simulink library "casper_library_communications"  (R2021a)
settings: Solver=ode45  StartTime=0.0  StopTime=10.0  RelTol=1e-3
undefined symbols (not defined in the file or in its folder): Down, Up
libraries: xbsIndex_r4 x292, casper_library_misc x6, xbsReplacements_r4 x6, xps_library x2
(part 1 of 2)
settings Model: Creator=mdexter  LastModifiedBy=jkocz
settings SolverCC: AlgebraicLoopSolver=TrustRegion
settings DataIOCC: LimitDataPoints=on  SaveFormat=Array  SignalLoggingSaveFormat=ModelDataLogs  ReturnWorkspaceOutputs=off
settings OptimizationCC: BlockReduction=off  BooleanDataType=off  ExpressionDepthLimit=2147483647  LifeSpan=inf
settings DebuggingCC: SaveWithParameterizedLinksMsg=none  UnderspecifiedInitializationDetection=Classic  MergeDetectMultiDrivingBlocksExec=none  SignalResolutionControl=TryResolveAllWithWarning  FcnCallInpInsideContextMsg=warning  StateNameClashWarn=warning  SFUnexpectedBacktrackingDiag=warning  SFNoUnconditionalDefaultTransitionDiag=warning  SFExecutionAtInitializationDiag=none  SFMachineParentedDataDiag=warning  ArithmeticOperatorsInVariantConditions=warning
settings HardwareCC: ProdBitPerPointer=32  ProdBitPerSizeT=32  ProdBitPerPtrDiffT=32  ProdLargestAtomicFloat=None  ProdIntDivRoundTo=Undefined  ProdEndianess=Unspecified  ProdWordSize=32  ProdHWDeviceType=32-bit Generic  TargetUnknown=on
settings ModelReferenceCC: PropagateSignalLabelsOutOfModel=off
settings SFSimCC: SimUseLocalCustomCode=off  CustomCodeUndefinedFunction=UseInterfaceOnly
settings RTWCC: RTWUseLocalCustomCode=off
settings CodeAppCC: StateflowObjectComments=on
settings GRTTargetCC: TargetLangStandard=C89/C90 (ANSI)  CombineOutputUpdateFcns=off  GRTInterface=on
settings ConfigComp: CovMetricSettings=dw  CovSaveCumulativeToWorkspaceVar=on  CovSaveSingleToWorkspaceVar=on  CovExternalEMLEnable=off

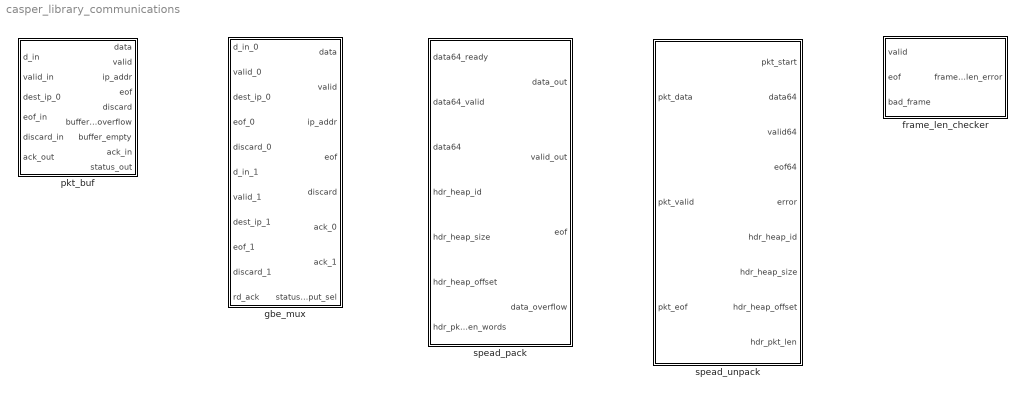
== system casper_library_communications ==
  frame_len_checker : Subsystem  Tag=casper:frame_len_checker  mask{frame_len=640 + 3 + 1}
      mask prompts: frame_len "Frame length (64-bit words):"
      mask help: Monitors valid, EOF and bad_frame signals in/from a 10Gbe core and outputs an error signal. Can be used to drive an error counter or latched as a flag.
  gbe_mux : Subsystem  mask(pkt_mux){}
      mask help: Merges two packet streams into one. Does round-robin arbitration.
  pkt_buf : Subsystem  mask(mux_packets){depth_data_bits=10, depth_hdr_bits=5}
      mask prompts: depth_data_bits "Depth contents (2^?)"; depth_hdr_bits "Maximum number of packets to buffer? (2^?)"
      mask help: This block allows you to buffer a 10GbE datastream.
      mask init:
      | fmtstr = sprintf('Max %d data words.\nMax %d pkts.', 2^depth_data_bits,2^depth_hdr_bits);
      | set_param(gcb, 'AttributesFormatString', fmtstr);
      settings: AttributesFormatString=|
      | Max 1024 data words.
      | Max 32 pkts.
  spead_pack : Subsystem  Tag=casper:spead_pack  mask(pkt_pack_mask){max_pkt_len_bits=10, header_ids=0x1600, 0x1234, header_ind_ids=0x1800, spead_msw=64, spead_lsw=40, spead_version=4, bytes_per_word=8}
      mask prompts: max_pkt_len_bits "Max pkt length, 2^? 64-bit words"; header_ids "SPEAD direct address IDs (decimal)"; header_ind_ids "SPEAD indirect address IDs (decimal)"; spead_msw "SPEAD Flavour (MSw)"; spead_lsw "SPEAD Flavour (LSw)"; spead_version "SPEAD version"; bytes_per_word "Word size, in bytes"
      mask help:
      | This block generates SPEAD-compliant packets from a datastream.
      |
      | Packets are created with a fixed header followed by a number of 64-bit items.
      |
      | Requires a 64-bit data stream.
      |
      | The data_ready signal is one cycle BEFORE valid data! Does not have to be with a valid signal either.
      mask init:
      | if floor(log2(bytes_per_word)) ~= log2(bytes_per_word)
      |     error('Bytes per word should be a power of two.');
      | end
      | 
      | spead_pack_init(gcb)
  spead_unpack : Subsystem  Tag=casper:spead_unpack  mask(spead_unpack_mask){max_pkt_len_bits=10, header_ids=0x1600, 0x1234, header_ind_ids=0x1800, spead_msw=64, spead_lsw=40, spead_version=4, combine_errors=on}
      mask prompts: max_pkt_len_bits "Max pkt length, 2^? 64-bit words"; header_ids "SPEAD direct header IDs (decimal)"; header_ind_ids "SPEAD indirect address IDs (decimal)"; spead_msw "SPEAD Flavour (MSw)"; spead_lsw "SPEAD Flavour (LSw)"; spead_version "SPEAD version"; combine_errors "Combine error flags"
      mask help: This block receives a 64-bit-word stream that contains a SPEAD stream. It checks the SPEAD headers are being correctly received. It presents the user with all headers on the first valid cycle of data along with a flag to indicate a header or packet-length error.
      mask init:
      | spead_unpack_init(gcb)

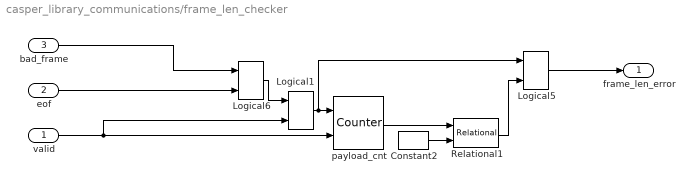
== system casper_library_communications/frame_len_checker ==
  valid : Inport
  eof : Inport  Port=2
  bad_frame : Inport  Port=3
  Constant2 : xbsIndex_r4/Constant  const=frame_len - 1  gui_display_data_type=Fixed-point  arith_type=Unsigned  n_bits=(ceil(log2(frame_len)))+1  bin_pt=0  preci_type=Single  exp_width=8  frac_width=24  explicit_period=on  period=1  equ=P=C  opselect=C  inp2=PCIN>>17  opr=+  inp1=P  carry=CIN  dbl_ovrd=off  block_type=constant
  Logical1 : xbsIndex_r4/Logical  logical_function=AND  inputs=2  en=off  latency=0  precision=Full  arith_type=Unsigned  n_bits=8  bin_pt=2  align_bp=on  dbl_ovrd=off  block_type=logical
      settings: xl_area=[0, 0, 0, 0, 0, 0, 0]
  Logical5 : xbsIndex_r4/Logical  logical_function=AND  inputs=2  en=off  latency=0  precision=Full  arith_type=Unsigned  n_bits=8  bin_pt=2  align_bp=on  dbl_ovrd=off  block_type=logical
      settings: xl_area=[0, 0, 0, 0, 0, 0, 0]
  Logical6 : xbsIndex_r4/Logical  logical_function=OR  inputs=2  en=off  latency=0  precision=Full  arith_type=Unsigned  n_bits=8  bin_pt=2  align_bp=on  dbl_ovrd=off  block_type=logical
      settings: xl_area=[0, 0, 0, 0, 0, 0, 0]
  Relational1 : xbsIndex_r4/Relational  mode=a!=b  op_type=Bool  en=off  latency=0  dbl_ovrd=off  block_type=relational
      settings: xl_area=[0, 0, 0, 0, 0, 0, 0]  block_version=10.1.3
  payload_cnt : xbsIndex_r4/Counter  cnt_type=Free Running  cnt_to=frame_len - 1  operation=Up  start_count=0  cnt_by_val=1  arith_type=Unsigned  n_bits=(ceil(log2(frame_len)))+1  bin_pt=0  load_pin=off  rst=on  en=on  explicit_period=off  period=1  use_behavioral_HDL=off  implementation=Fabric  use_rpm=on  dbl_ovrd=off  block_type=counter
      settings: xl_area=[0, 0, 0, 0, 0, 0, 0]
  frame_len_error : Outport  VectorParamsAs1DForOutWhenUnconnected=off
  wires:
  Logical1/1 -> Logical5/1, payload_cnt/1
  eof/1 -> Logical6/2
  Relational1/1 -> Logical5/2
  payload_cnt/1 -> Relational1/1
  Constant2/1 -> Relational1/2
  bad_frame/1 -> Logical6/1
  valid/1 -> Logical1/2, payload_cnt/2
  Logical6/1 -> Logical1/1
  Logical5/1 -> frame_len_error/1

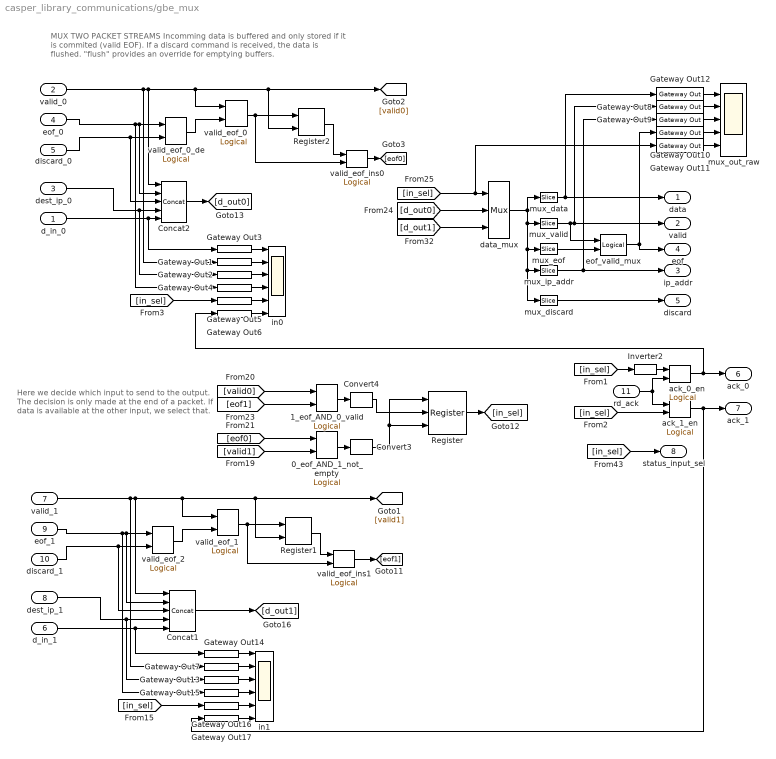
== system casper_library_communications/gbe_mux ==
  note: MUX TWO PACKET STREAMS
      | Incomming data is buffered and only stored if it is commited (valid EOF).
      | If a discard command is received, the data is flushed.
      | "flush" provides an override for emptying buffers.
  note: Here we decide which input
      | to send to the output.
      | The decision is only made at the end of a packet.
      | If data is available at the other input,
      | we select that.
  d_in_0 : Inport
  valid_0 : Inport  Port=2
  dest_ip_0 : Inport  Port=3
  eof_0 : Inport  Port=4
  discard_0 : Inport  Port=5
  d_in_1 : Inport  Port=6
  valid_1 : Inport  Port=7
  dest_ip_1 : Inport  Port=8
  eof_1 : Inport  Port=9
  discard_1 : Inport  Port=10
  rd_ack : Inport  Port=11
  0_eof_AND_1_not_empty : xbsIndex_r4/Logical  logical_function=AND  inputs=2  en=off  latency=0  precision=Full  arith_type=Unsigned  n_bits=8  bin_pt=2  align_bp=on  dbl_ovrd=off  block_type=logical
      settings: xl_area=[0, 0, 0, 0, 0, 0, 0]
  1_eof_AND_0_valid : xbsIndex_r4/Logical  logical_function=AND  inputs=2  en=off  latency=0  precision=Full  arith_type=Unsigned  n_bits=8  bin_pt=2  align_bp=on  dbl_ovrd=off  block_type=logical
      settings: xl_area=[0, 0, 0, 0, 0, 0, 0]
  Concat1 : xbsIndex_r4/Concat  num_inputs=5  dbl_ovrd=off  block_type=concat
      settings: block_version=10.1.3
  Concat2 : xbsIndex_r4/Concat  num_inputs=5  dbl_ovrd=off  block_type=concat
      settings: block_version=10.1.3
  Convert3 : xbsIndex_r4/Convert  gui_display_data_type=Fixed-point  arith_type=Boolean  n_bits=8  bin_pt=6  float_type=Single  exp_bits=8  fraction_bits=24  quantization=Truncate  overflow=Wrap  en=off  latency=0  pipeline=off  dbl_ovrd=off  block_type=convert
      settings: xl_area=[0, 0, 0, 0, 0, 0, 0]  block_version=10.1.3
  Convert4 : xbsIndex_r4/Convert  gui_display_data_type=Fixed-point  arith_type=Boolean  n_bits=8  bin_pt=6  float_type=Single  exp_bits=8  fraction_bits=24  quantization=Truncate  overflow=Wrap  en=off  latency=0  pipeline=off  dbl_ovrd=off  block_type=convert
      settings: xl_area=[0, 0, 0, 0, 0, 0, 0]  block_version=10.1.3
  Gateway Out{1..17} (17 alike) : xbsIndex_r4/Gateway Out  inherit_from_input=off  hdl_port=off  rows=1  columns=1  UseAsDAC=off  DACChannel='1'  interface=None  automatic_assignment=on  address_offset=hex2dec('00')  intf_name=''  intf_description=''  timing_constraint=None  locs_specified=off  LOCs={}  io_standard={}  block_type=gatewayout
      settings: infoedit="Gateway out block.  Converts Xilinx fixed point inputs into ouputs of type Simulink integer, double, or fixed point.<P><P>Hardware notes:  In hardware these blocks become top level output ports or are discarded, depending on how they are configured."  xl_area=[0, 0, 0, 0, 0, 0, 0]  block_version=10.1.3
  Inverter2 : xbsIndex_r4/Inverter  en=off  latency=0  dbl_ovrd=off  block_type=inv
      settings: xl_area=[0, 0, 0, 0, 0, 0, 0]
  Register : xbsIndex_r4/Register  init=0  rst=on  en=on  dbl_ovrd=off  block_type=register
      settings: xl_area=[0, 0, 0, 0, 0, 0, 0]
  Register1 : xbsIndex_r4/Register  init=1  rst=off  en=on  dbl_ovrd=off  block_type=register
      settings: xl_area=[0, 0, 0, 0, 0, 0, 0]
  Register2 : xbsIndex_r4/Register  init=0  rst=off  en=on  dbl_ovrd=off  block_type=register
      settings: xl_area=[0, 0, 0, 0, 0, 0, 0]
  ack_0_en : xbsIndex_r4/Logical  logical_function=AND  inputs=2  en=off  latency=0  precision=Full  arith_type=Unsigned  n_bits=8  bin_pt=2  align_bp=on  dbl_ovrd=off  block_type=logical
      settings: xl_area=[0, 0, 0, 0, 0, 0, 0]
  ack_1_en : xbsIndex_r4/Logical  logical_function=AND  inputs=2  en=off  latency=0  precision=Full  arith_type=Unsigned  n_bits=8  bin_pt=2  align_bp=on  dbl_ovrd=off  block_type=logical
      settings: xl_area=[0, 0, 0, 0, 0, 0, 0]
  data_mux : xbsIndex_r4/Mux  inputs=2  en=off  latency=0  precision=Full  arith_type="Signed  (2's comp)"  n_bits=8  bin_pt=2  quantization=Truncate  overflow=Wrap  dbl_ovrd=off  block_type=mux
      settings: xl_area=[0, 0, 0, 0, 0, 0, 0]
  eof_valid_mux : xbsIndex_r4/Logical  logical_function=AND  inputs=2  en=off  latency=0  precision=Full  arith_type=Unsigned  n_bits=8  bin_pt=2  align_bp=on  dbl_ovrd=off  block_type=logical
      settings: xl_area=[0, 0, 0, 0, 0, 0, 0]
  in0 : Scope  NumInputPorts=6
  in1 : Scope  NumInputPorts=6
  mux_data : xbsIndex_r4/Slice  nbits=64  boolean_output=off  mode=Lower Bit Location + Width  bit1=33  base1=LSB of Input  bit0=0  base0=LSB of Input  dbl_ovrd=off  block_type=slice
      settings: infoedit="Extracts a given range of bits from each input sample and presents it at the output.  The output type is ordinarily unsigned with binary point at zero, but can be Boolean when the slice is one bit wide.<P><P>Hardware notes: In hardware this block costs nothing."  block_version=10.1.3
  mux_discard : xbsIndex_r4/Slice  nbits=1  boolean_output=on  mode=Lower Bit Location + Width  bit1=0  base1=MSB of Input  bit0=96  base0=LSB of Input  dbl_ovrd=off  block_type=slice
      settings: infoedit="Extracts a given range of bits from each input sample and presents it at the output.  The output type is ordinarily unsigned with binary point at zero, but can be Boolean when the slice is one bit wide.<P><P>Hardware notes: In hardware this block costs nothing."  block_version=10.1.3
  mux_eof : xbsIndex_r4/Slice  nbits=1  boolean_output=on  mode=Upper Bit Location + Width  bit1=97  base1=LSB of Input  bit0=0  base0=LSB of Input  dbl_ovrd=off  block_type=slice
      settings: infoedit="Extracts a given range of bits from each input sample and presents it at the output.  The output type is ordinarily unsigned with binary point at zero, but can be Boolean when the slice is one bit wide.<P><P>Hardware notes: In hardware this block costs nothing."  block_version=10.1.3
  mux_ip_addr : xbsIndex_r4/Slice  nbits=32  boolean_output=off  mode=Lower Bit Location + Width  bit1=0  base1=MSB of Input  bit0=64  base0=LSB of Input  dbl_ovrd=off  block_type=slice
      settings: infoedit="Extracts a given range of bits from each input sample and presents it at the output.  The output type is ordinarily unsigned with binary point at zero, but can be Boolean when the slice is one bit wide.<P><P>Hardware notes: In hardware this block costs nothing."  block_version=10.1.3
  mux_out_raw : Scope  NumInputPorts=5
  mux_valid : xbsIndex_r4/Slice  nbits=1  boolean_output=on  mode=Lower Bit Location + Width  bit1=0  base1=MSB of Input  bit0=98  base0=LSB of Input  dbl_ovrd=off  block_type=slice
      settings: infoedit="Extracts a given range of bits from each input sample and presents it at the output.  The output type is ordinarily unsigned with binary point at zero, but can be Boolean when the slice is one bit wide.<P><P>Hardware notes: In hardware this block costs nothing."  block_version=10.1.3
  valid_eof_0 : xbsIndex_r4/Logical  logical_function=AND  inputs=2  en=off  latency=0  precision=Full  arith_type=Unsigned  n_bits=8  bin_pt=2  align_bp=on  dbl_ovrd=off  block_type=logical
      settings: xl_area=[0, 0, 0, 0, 0, 0, 0]
  valid_eof_0_de : xbsIndex_r4/Logical  logical_function=OR  inputs=2  en=off  latency=0  precision=Full  arith_type=Unsigned  n_bits=8  bin_pt=2  align_bp=on  dbl_ovrd=off  block_type=logical
      settings: xl_area=[0, 0, 0, 0, 0, 0, 0]
  valid_eof_1 : xbsIndex_r4/Logical  logical_function=AND  inputs=2  en=off  latency=0  precision=Full  arith_type=Unsigned  n_bits=8  bin_pt=2  align_bp=on  dbl_ovrd=off  block_type=logical
      settings: xl_area=[0, 0, 0, 0, 0, 0, 0]
  valid_eof_2 : xbsIndex_r4/Logical  logical_function=OR  inputs=2  en=off  latency=0  precision=Full  arith_type=Unsigned  n_bits=8  bin_pt=2  align_bp=on  dbl_ovrd=off  block_type=logical
      settings: xl_area=[0, 0, 0, 0, 0, 0, 0]
  valid_eof_ins0 : xbsIndex_r4/Logical  logical_function=OR  inputs=2  en=off  latency=0  precision=Full  arith_type=Unsigned  n_bits=8  bin_pt=2  align_bp=on  dbl_ovrd=off  block_type=logical
      settings: xl_area=[0, 0, 0, 0, 0, 0, 0]
  valid_eof_ins1 : xbsIndex_r4/Logical  logical_function=OR  inputs=2  en=off  latency=0  precision=Full  arith_type=Unsigned  n_bits=8  bin_pt=2  align_bp=on  dbl_ovrd=off  block_type=logical
      settings: xl_area=[0, 0, 0, 0, 0, 0, 0]
  data : Outport  VectorParamsAs1DForOutWhenUnconnected=off
  valid : Outport  Port=2  VectorParamsAs1DForOutWhenUnconnected=off
  ip_addr : Outport  Port=3  VectorParamsAs1DForOutWhenUnconnected=off
  eof : Outport  Port=4  VectorParamsAs1DForOutWhenUnconnected=off
  discard : Outport  Port=5  VectorParamsAs1DForOutWhenUnconnected=off
  ack_0 : Outport  Port=6  VectorParamsAs1DForOutWhenUnconnected=off
  ack_1 : Outport  Port=7  VectorParamsAs1DForOutWhenUnconnected=off
  status_input_sel : Outport  Port=8  VectorParamsAs1DForOutWhenUnconnected=off
  wires:
  valid_eof_ins0/1 -> [eof0]
  Register2/1 -> valid_eof_ins0/1
  Register1/1 -> valid_eof_ins1/1
  valid_eof_ins1/1 -> [eof1]
  Gateway Out17/1 -> in1/6
  Gateway Out6/1 -> in0/6
  mux_discard/1 -> discard/1
  d_in_0/1 -> Concat2/5, Gateway Out3/1
  dest_ip_0/1 -> Gateway Out2/1, Concat2/4
  valid_eof_0_de/1 -> valid_eof_0/2
  discard_0/1 -> Concat2/3, valid_eof_0_de/2
  eof_0/1 -> Gateway Out4/1, Concat2/2, valid_eof_0_de/1
  Gateway Out5/1 -> in0/5
  [in_sel] -> Gateway Out5/1
  Gateway Out4/1 -> in0/4
  Gateway Out2/1 -> in0/3
  Gateway Out1/1 -> in0/2
  Gateway Out3/1 -> in0/1
  Concat2/1 -> [d_out0]
  valid_eof_0/1 -> valid_eof_ins0/2, Register2/1
  valid_0/1 -> Gateway Out1/1, Concat2/1, [valid0], Register2/2, valid_eof_0/1
  d_in_1/1 -> Gateway Out14/1, Concat1/5
  dest_ip_1/1 -> Gateway Out13/1, Concat1/4
  [in_sel] -> Inverter2/1
  Inverter2/1 -> ack_0_en/1
  [in_sel] -> ack_1_en/2
  rd_ack/1 -> ack_1_en/1, ack_0_en/2
  ack_1_en/1 -> Gateway Out17/1, ack_1/1
  ack_0_en/1 -> Gateway Out6/1, ack_0/1
  valid_eof_2/1 -> valid_eof_1/2
  discard_1/1 -> Concat1/3, valid_eof_2/2
  eof_1/1 -> Gateway Out15/1, Concat1/2, valid_eof_2/1
  Gateway Out16/1 -> in1/5
  [in_sel] -> Gateway Out16/1
  Register/1 -> [in_sel]
  Gateway Out11/1 -> mux_out_raw/5
  Gateway Out15/1 -> in1/4
  Gateway Out13/1 -> in1/3
  Gateway Out7/1 -> in1/2
  Gateway Out14/1 -> in1/1
  mux_eof/1 -> eof_valid_mux/2
  eof_valid_mux/1 -> Gateway Out10/1, eof/1
  mux_ip_addr/1 -> Gateway Out9/1, ip_addr/1
  mux_valid/1 -> Gateway Out8/1, valid/1, eof_valid_mux/1
  mux_data/1 -> data/1, Gateway Out12/1
  data_mux/1 -> mux_data/1, mux_valid/1, mux_eof/1, mux_discard/1, mux_ip_addr/1
  Concat1/1 -> [d_out1]
  valid_eof_1/1 -> valid_eof_ins1/2, Register1/1
  [in_sel] -> status_input_sel/1
  [d_out1] -> data_mux/3
  [d_out0] -> data_mux/2
  [in_sel] -> Gateway Out11/1, data_mux/1
  [eof1] -> 1_eof_AND_0_valid/2
  [eof0] -> 0_eof_AND_1_not_empty/1
  [valid0] -> 1_eof_AND_0_valid/1
  [valid1] -> 0_eof_AND_1_not_empty/2
  Gateway Out10/1 -> mux_out_raw/4
  Gateway Out9/1 -> mux_out_raw/3
  Gateway Out8/1 -> mux_out_raw/2
  Gateway Out12/1 -> mux_out_raw/1
  Convert4/1 -> Register/2
  Convert3/1 -> Register/1, Register/3
  1_eof_AND_0_valid/1 -> Convert4/1
  0_eof_AND_1_not_empty/1 -> Convert3/1
  valid_1/1 -> Gateway Out7/1, Concat1/1, [valid1], Register1/2, valid_eof_1/1

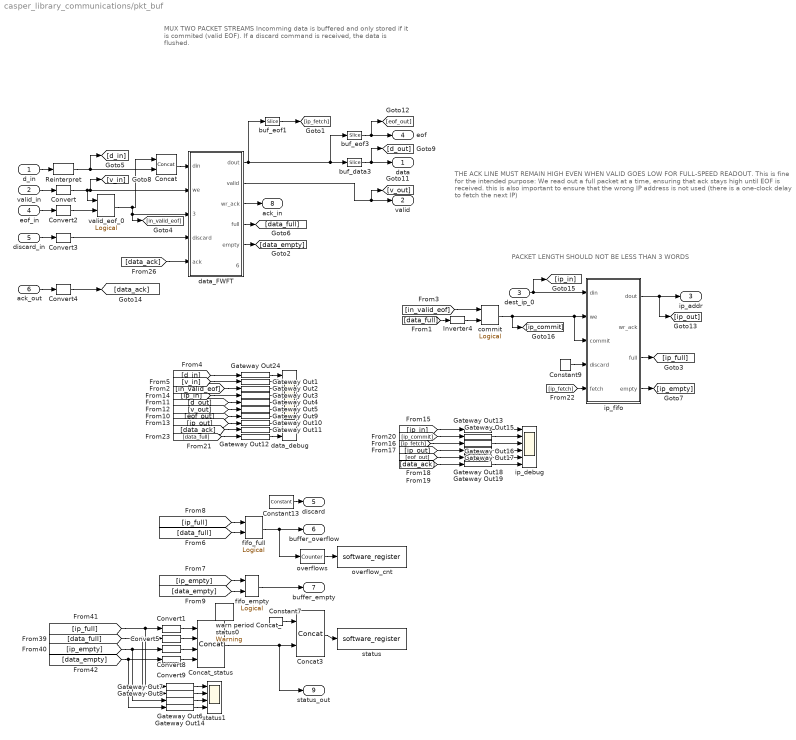
== system casper_library_communications/pkt_buf ==
  note: PACKET LENGTH SHOULD NOT BE LESS THAN 3 WORDS
  note: THE ACK LINE MUST REMAIN HIGH EVEN WHEN VALID GOES LOW FOR FULL-SPEED READOUT.
      |
      | This is fine for the intended purpose:
      | We read out a full packet at a time, ensuring that ack stays high until EOF is received.
      |
      | this is also important to ensure that the wrong IP address is not used
      | (there is a one-clock delay to fetch the next IP)
  note: MUX TWO PACKET STREAMS
      | Incomming data is buffered and only stored if it is commited (valid EOF).
      | If a discard command is received, the data is flushed.
  d_in : Inport
  valid_in : Inport  Port=2
  dest_ip_0 : Inport  Port=3
  eof_in : Inport  Port=4
  discard_in : Inport  Port=5
  ack_out : Inport  Port=6
  Concat : xbsIndex_r4/Concat  num_inputs=2  dbl_ovrd=off  block_type=concat
      settings: block_version=10.1.3
  Concat3 : xbsIndex_r4/Concat  num_inputs=2  dbl_ovrd=off  block_type=concat
      settings: block_version=10.1.3
  Concat_status : xbsIndex_r4/Concat  num_inputs=4  dbl_ovrd=off  block_type=concat
      settings: block_version=10.1.3
  Constant13 : xbsIndex_r4/Constant  const=0  gui_display_data_type=Fixed-point  arith_type=Boolean  n_bits=1  bin_pt=0  preci_type=Single  exp_width=8  frac_width=24  explicit_period=on  period=1  equ=P=C  opselect=C  inp2=PCIN>>17  opr=+  inp1=P  carry=CIN  dbl_ovrd=off  block_type=constant
  Constant7 : xbsIndex_r4/Constant  const=0  gui_display_data_type=Fixed-point  arith_type=Unsigned  n_bits=32-9  bin_pt=0  preci_type=Single  exp_width=8  frac_width=24  explicit_period=on  period=1  equ=P=C  opselect=C  inp2=PCIN>>17  opr=+  inp1=P  carry=CIN  dbl_ovrd=off  block_type=constant
  Constant9 : xbsIndex_r4/Constant  const=0  gui_display_data_type=Fixed-point  arith_type=Boolean  n_bits=1  bin_pt=0  preci_type=Single  exp_width=8  frac_width=24  explicit_period=on  period=1  equ=P=C  opselect=C  inp2=PCIN>>17  opr=+  inp1=P  carry=CIN  dbl_ovrd=off  block_type=constant
  Convert{,2..4} (4 alike) : xbsIndex_r4/Convert  gui_display_data_type=Fixed-point  arith_type=Boolean  n_bits=8  bin_pt=6  float_type=Single  exp_bits=8  fraction_bits=24  quantization=Truncate  overflow=Wrap  en=off  latency=0  pipeline=off  dbl_ovrd=off  block_type=convert
      settings: xl_area=[0, 0, 0, 0, 0, 0, 0]  block_version=10.1.3
  Convert{1,5,8..9} (4 alike) : xbsIndex_r4/Convert  gui_display_data_type=Fixed-point  arith_type=Unsigned  n_bits=1  bin_pt=0  float_type=Single  exp_bits=8  fraction_bits=24  quantization=Truncate  overflow=Wrap  en=off  latency=0  pipeline=off  dbl_ovrd=off  block_type=convert
      settings: xl_area=[0, 0, 0, 0, 0, 0, 0]  block_version=10.1.3
  Gateway Out{1..5,9..13,15..19,24} (16 alike) : xbsIndex_r4/Gateway Out  inherit_from_input=off  hdl_port=off  rows=1  columns=1  UseAsDAC=off  DACChannel='1'  interface=None  automatic_assignment=on  address_offset=hex2dec('00')  intf_name=''  intf_description=''  timing_constraint=None  locs_specified=off  LOCs={}  io_standard={}  block_type=gatewayout
      settings: infoedit="Gateway out block.  Converts Xilinx fixed point inputs into ouputs of type Simulink integer, double, or fixed point.<P><P>Hardware notes:  In hardware these blocks become top level output ports or are discarded, depending on how they are configured."  xl_area=[0, 0, 0, 0, 0, 0, 0]  block_version=10.1.3
  Gateway Out{6..8,14} (4 alike) : xbsIndex_r4/Gateway Out  inherit_from_input=off  hdl_port=on  rows=1  columns=1  UseAsDAC=off  DACChannel='1'  interface=None  automatic_assignment=on  address_offset=hex2dec('00')  intf_name=''  intf_description=''  timing_constraint=None  locs_specified=off  LOCs={}  io_standard={}  block_type=gatewayout
      settings: infoedit="Gateway out block.  Converts Xilinx fixed point inputs into ouputs of type Simulink integer, double, or fixed point.<P><P>Hardware notes:  In hardware these blocks become top level output ports or are discarded, depending on how they are configured."  xl_area=[0, 0, 0, 0, 0, 0, 0]  block_version=10.1.3
  Inverter4 : xbsIndex_r4/Inverter  en=off  latency=0  dbl_ovrd=off  block_type=inv
      settings: xl_area=[0, 0, 0, 0, 0, 0, 0]
  Reinterpret : xbsIndex_r4/Reinterpret  force_arith_type=on  arith_type=Unsigned  force_bin_pt=on  bin_pt=0  block_type=reinterpret
      settings: infoedit="Changes signal type without altering the binary representation.   You can changed the signal between signed and unsigned, and relocate the binary point.<P><P>Hardware notes: In hardware this block costs nothing.<P><P>Example:  Suppose the input is 6 bits wide, signed, with 2 fractional bits, and the output is forced to unsigned with 0 fractional bits.  Then an input of -2.0 (1110.00 in binary 2's complement) becomes an output of 56 (111000 in binary)."  block_version=10.1.3
  buf_data3 : xbsIndex_r4/Slice  nbits=64  boolean_output=off  mode=Lower Bit Location + Width  bit1=33  base1=LSB of Input  bit0=0  base0=LSB of Input  dbl_ovrd=off  block_type=slice
      settings: infoedit="Extracts a given range of bits from each input sample and presents it at the output.  The output type is ordinarily unsigned with binary point at zero, but can be Boolean when the slice is one bit wide.<P><P>Hardware notes: In hardware this block costs nothing."  block_version=10.1.3
  buf_eof1 : xbsIndex_r4/Slice  nbits=1  boolean_output=on  mode=Upper Bit Location + Width  bit1=64  base1=LSB of Input  bit0=0  base0=LSB of Input  dbl_ovrd=off  block_type=slice
      settings: infoedit="Extracts a given range of bits from each input sample and presents it at the output.  The output type is ordinarily unsigned with binary point at zero, but can be Boolean when the slice is one bit wide.<P><P>Hardware notes: In hardware this block costs nothing."  block_version=10.1.3
  buf_eof3 : xbsIndex_r4/Slice  nbits=1  boolean_output=on  mode=Upper Bit Location + Width  bit1=64  base1=LSB of Input  bit0=0  base0=LSB of Input  dbl_ovrd=off  block_type=slice
      settings: infoedit="Extracts a given range of bits from each input sample and presents it at the output.  The output type is ordinarily unsigned with binary point at zero, but can be Boolean when the slice is one bit wide.<P><P>Hardware notes: In hardware this block costs nothing."  block_version=10.1.3
  commit : xbsIndex_r4/Logical  logical_function=AND  inputs=2  en=off  latency=0  precision=Full  arith_type=Unsigned  n_bits=8  bin_pt=2  align_bp=on  dbl_ovrd=off  block_type=logical
      settings: xl_area=[0, 0, 0, 0, 0, 0, 0]
  data_FWFT : Subsystem  mask{depth_bits=depth_data_bits, burst_bits=depth_data_bits-1}
      mask prompts: depth_bits "Fifo Depth (2^?):"; burst_bits "Issue almost full warning when (2^?) from full"
      mask help: A rollback fifo behaves as a normal fifo, except that data which are written in have to be "committed" before they become available for readout. Moreover, any data which are written in and have not been committed can be "discarded", and will never be made available for readout.
      mask init:
      | fmtstr = sprintf('Depth: %d', 2^depth_bits);
      | set_param(gcb, 'AttributesFormatString', fmtstr);
      settings: AttributesFormatString=Depth: 1024
  data_debug : Scope  NumInputPorts=10
  fifo_empty : xbsIndex_r4/Logical  logical_function=AND  inputs=2  en=off  latency=0  precision=Full  arith_type=Unsigned  n_bits=8  bin_pt=2  align_bp=on  dbl_ovrd=off  block_type=logical
      settings: xl_area=[0, 0, 0, 0, 0, 0, 0]
  fifo_full : xbsIndex_r4/Logical  logical_function=OR  inputs=2  en=off  latency=0  precision=Full  arith_type=Unsigned  n_bits=8  bin_pt=2  align_bp=on  dbl_ovrd=off  block_type=logical
      settings: xl_area=[0, 0, 0, 0, 0, 0, 0]
  ip_debug : Scope  NumInputPorts=6
  ip_fifo : Subsystem  mask{depth_bits=depth_hdr_bits}
      mask prompts: depth_bits "Fifo Depth (2^?):"
      mask help: A rollback fifo behaves as a normal fifo, except that data which are written in have to be "committed" before they become available for readout. Moreover, any data which are written in and have not been committed can be "discarded", and will never be made available for readout.
      mask init:
      | fmtstr = sprintf('Depth: %d', 2^depth_bits);
      | set_param(gcb, 'AttributesFormatString', fmtstr);
      settings: AttributesFormatString=Depth: 32
  overflow_cnt : xps_library/Memory/software_register  Tag=xps:sw_reg  io_dir=To Processor  io_delay=0  init_val=0  sample_period=1  names=reg  bitwidths=32  bin_pts=0  arith_types=0  sim_port=on  show_format=off
      settings: AttributesFormatString=1output  SourceProductName=CASPER XPS Blockset
  overflows : xbsIndex_r4/Counter  cnt_type=Free Running  cnt_to=Inf  operation=Up  start_count=0  cnt_by_val=1  arith_type=Unsigned  n_bits=32  bin_pt=0  load_pin=off  rst=off  en=on  explicit_period=off  period=1  use_behavioral_HDL=off  implementation=Fabric  use_rpm=on  dbl_ovrd=off  block_type=counter
      settings: xl_area=[0, 0, 0, 0, 0, 0, 0]
  status : xps_library/Memory/software_register  Tag=xps:sw_reg  io_dir=To Processor  io_delay=0  init_val=0  sample_period=1  names=reg  bitwidths=32  bin_pts=0  arith_types=0  sim_port=on  show_format=off
      settings: AttributesFormatString=1output  SourceProductName=CASPER XPS Blockset
  status1 : Scope  NumInputPorts=4
  valid_eof_0 : xbsIndex_r4/Logical  logical_function=AND  inputs=2  en=off  latency=0  precision=Full  arith_type=Unsigned  n_bits=8  bin_pt=2  align_bp=on  dbl_ovrd=off  block_type=logical
      settings: xl_area=[0, 0, 0, 0, 0, 0, 0]
  warn period Concat_status0 : xbsReplacements_r4/Warning  period=1
  data : Outport  VectorParamsAs1DForOutWhenUnconnected=off
  valid : Outport  Port=2  VectorParamsAs1DForOutWhenUnconnected=off
  ip_addr : Outport  Port=3  VectorParamsAs1DForOutWhenUnconnected=off
  eof : Outport  Port=4  VectorParamsAs1DForOutWhenUnconnected=off
  discard : Outport  Port=5  VectorParamsAs1DForOutWhenUnconnected=off
  buffer_overflow : Outport  Port=6  VectorParamsAs1DForOutWhenUnconnected=off
  buffer_empty : Outport  Port=7  VectorParamsAs1DForOutWhenUnconnected=off
  ack_in : Outport  Port=8  VectorParamsAs1DForOutWhenUnconnected=off
  status_out : Outport  Port=9  VectorParamsAs1DForOutWhenUnconnected=off
  wires:
  [data_full] -> Gateway Out12/1
  Gateway Out12/1 -> data_debug/10
  Convert4/1 -> [data_ack]
  Convert3/1 -> data_FWFT/4(discard)
  Convert2/1 -> valid_eof_0/2
  Convert/1 -> data_FWFT/2(we), [v_in], valid_eof_0/1
  Reinterpret/1 -> [d_in], Concat/2
  [ip_fetch] -> ip_fifo/5(fetch)
  buf_eof1/1 -> [ip_fetch]
  [data_ack] -> Gateway Out11/1
  Gateway Out11/1 -> data_debug/9
  [data_ack] -> data_FWFT/5(ack)
  [ip_fetch] -> Gateway Out16/1
  [data_full] -> Inverter4/1
  [ip_commit] -> Gateway Out15/1
  [data_ack] -> Gateway Out19/1
  ack_out/1 -> Convert4/1
  [eof_out] -> Gateway Out18/1
  [ip_out] -> Gateway Out17/1
  [ip_in] -> Gateway Out13/1
  [in_valid_eof] -> Gateway Out2/1
  [v_in] -> Gateway Out1/1
  [d_in] -> Gateway Out24/1
  [ip_in] -> Gateway Out3/1
  [d_out] -> Gateway Out4/1
  [v_out] -> Gateway Out5/1
  [eof_out] -> Gateway Out9/1
  [ip_out] -> Gateway Out10/1
  Gateway Out10/1 -> data_debug/8
  Convert9/1 -> Concat_status/4
  Convert8/1 -> Concat_status/3
  Convert5/1 -> Concat_status/2
  Convert1/1 -> Concat_status/1
  Gateway Out14/1 -> status1/4
  Gateway Out6/1 -> status1/3
  Gateway Out8/1 -> status1/2
  Gateway Out7/1 -> status1/1
  [in_valid_eof] -> commit/1
  buf_eof3/1 -> [eof_out], eof/1
  buf_data3/1 -> [d_out], data/1
  data_FWFT/5(empty) -> [data_empty]
  Gateway Out19/1 -> ip_debug/6
  Gateway Out9/1 -> data_debug/7
  Gateway Out5/1 -> data_debug/6
  Gateway Out4/1 -> data_debug/5
  Gateway Out18/1 -> ip_debug/5
  Gateway Out17/1 -> ip_debug/4
  Gateway Out16/1 -> ip_debug/3
  Gateway Out15/1 -> ip_debug/2
  Gateway Out13/1 -> ip_debug/1
  Gateway Out3/1 -> data_debug/4
  Gateway Out2/1 -> data_debug/3
  Gateway Out1/1 -> data_debug/2
  Gateway Out24/1 -> data_debug/1
  overflows/1 -> overflow_cnt/1
  Constant9/1 -> ip_fifo/4(discard)
  ip_fifo/1(dout) -> [ip_out], ip_addr/1
  data_FWFT/2(valid) -> [v_out], valid/1
  data_FWFT/1(dout) -> buf_data3/1, buf_eof3/1, buf_eof1/1
  valid_eof_0/1 -> data_FWFT/3(commit), [in_valid_eof], Concat/1
  Inverter4/1 -> commit/2
  ip_fifo/4(empty) -> [ip_empty]
  data_FWFT/3(wr_ack) -> ack_in/1
  eof_in/1 -> Convert2/1
  dest_ip_0/1 -> [ip_in], ip_fifo/1(din)
  valid_in/1 -> Convert/1
  d_in/1 -> Reinterpret/1
  commit/1 -> [ip_commit], ip_fifo/2(we), ip_fifo/3(commit)
  ip_fifo/3(full) -> [ip_full]
  data_FWFT/4(full) -> [data_full]
  Concat/1 -> data_FWFT/1(din)
  discard_in/1 -> Convert3/1
  Constant7/1 -> Concat3/1
  Concat3/1 -> status/1
  Concat_status/1 -> status_out/1, Concat3/2
  [data_empty] -> Gateway Out14/1, Convert9/1
  [ip_empty] -> Gateway Out6/1, Convert8/1
  [data_full] -> Convert5/1, Gateway Out8/1
  [ip_full] -> Gateway Out7/1, Convert1/1
  [data_full] -> fifo_full/2
  [ip_full] -> fifo_full/1
  [data_empty] -> fifo_empty/2
  [ip_empty] -> fifo_empty/1
  fifo_empty/1 -> buffer_empty/1
  fifo_full/1 -> overflows/1, buffer_overflow/1
  Constant13/1 -> discard/1

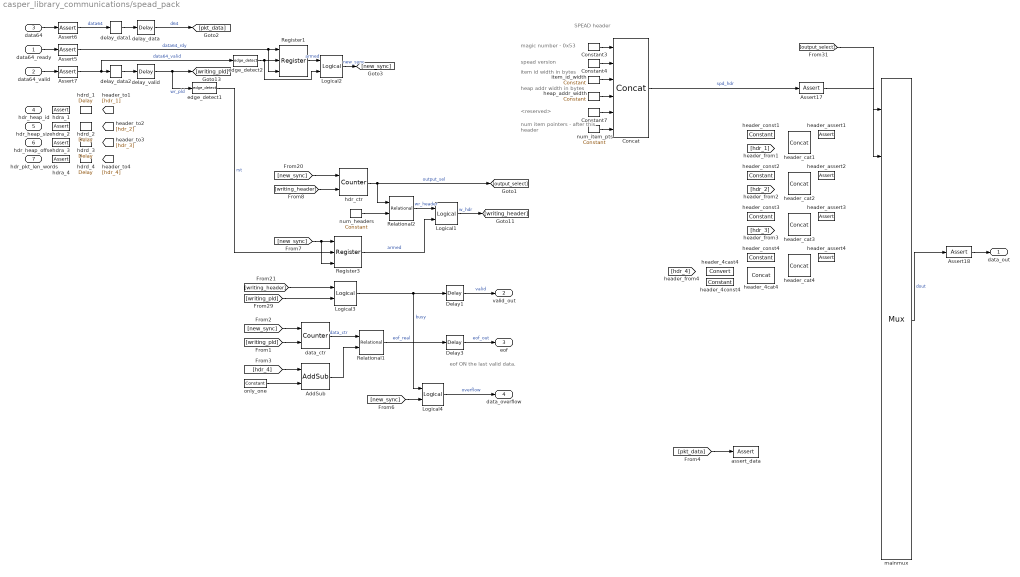
== system casper_library_communications/spead_pack ==
  note: eof ON the last valid data.
  note: SPEAD header
  note: magic number - 0x53
  note: spead version
  note: item id width in bytes
  note: heap addr width in bytes
  note: <reserved>
  note: num item pointers -
      | after this header
  data64_ready : Inport
  data64_valid : Inport  Port=2
  data64 : Inport  Port=3
  hdr_heap_id : Inport  Port=4
  hdr_heap_size : Inport  Port=5
  hdr_heap_offset : Inport  Port=6
  hdr_pkt_len_words : Inport  Port=7
  AddSub : xbsIndex_r4/AddSub  mode=Subtraction  use_carryin=off  use_carryout=off  en=off  latency=0  precision=Full  arith_type=Unsigned  n_bits=16  bin_pt=14  quantization=Truncate  overflow=Wrap  use_behavioral_HDL=off  hw_selection=Fabric  pipelined=off  dbl_ovrd=off  block_type=addsub
  Assert17 : xbsIndex_r4/Assert  assert_type=on  type_source=Explicitly  gui_display_data_type=Fixed-point  arith_type=Unsigned  n_bits=64  bin_pt=0  preci_type=Single  exp_width=8  frac_width=24  assert_rate=off  rate_source=Explicitly  period=1  output_port=on  block_type=assert
  Assert18 : xbsIndex_r4/Assert  assert_type=on  type_source=Explicitly  gui_display_data_type=Fixed-point  arith_type=Unsigned  n_bits=spead_msw  bin_pt=0  preci_type=Single  exp_width=8  frac_width=24  assert_rate=off  rate_source=Explicitly  period=1  output_port=on  block_type=assert
  Assert5 : xbsIndex_r4/Assert  assert_type=on  type_source=Explicitly  gui_display_data_type=Fixed-point  arith_type=Boolean  n_bits=64  bin_pt=0  preci_type=Single  exp_width=8  frac_width=24  assert_rate=off  rate_source=Explicitly  period=1  output_port=on  block_type=assert
      settings: block_version=10.1.3
  Assert6 : xbsIndex_r4/Assert  assert_type=on  type_source=Explicitly  gui_display_data_type=Fixed-point  arith_type=Unsigned  n_bits=spead_msw  bin_pt=0  preci_type=Single  exp_width=8  frac_width=24  assert_rate=off  rate_source=Explicitly  period=1  output_port=on  block_type=assert
      settings: block_version=10.1.3
  Assert7 : xbsIndex_r4/Assert  assert_type=on  type_source=Explicitly  gui_display_data_type=Boolean  arith_type=Boolean  n_bits=64  bin_pt=0  preci_type=Single  exp_width=8  frac_width=24  assert_rate=off  rate_source=Explicitly  period=1  output_port=on  block_type=assert
      settings: block_version=10.1.3
  Concat : xbsIndex_r4/Concat  num_inputs=6  dbl_ovrd=off  block_type=concat
      settings: block_version=10.1.3
  Constant3 : xbsIndex_r4/Constant  const=83  gui_display_data_type=Fixed-point  arith_type=Unsigned  n_bits=8  bin_pt=0  preci_type=Single  exp_width=8  frac_width=24  explicit_period=on  period=1  equ=P=C  opselect=C  inp2=PCIN>>17  opr=+  inp1=P  carry=CIN  dbl_ovrd=off  block_type=constant
  Constant4 : xbsIndex_r4/Constant  const=spead_version  gui_display_data_type=Fixed-point  arith_type=Unsigned  n_bits=8  bin_pt=0  preci_type=Single  exp_width=8  frac_width=24  explicit_period=on  period=1  equ=P=C  opselect=C  inp2=PCIN>>17  opr=+  inp1=P  carry=CIN  dbl_ovrd=off  block_type=constant
  Constant7 : xbsIndex_r4/Constant  const=0  gui_display_data_type=Fixed-point  arith_type=Unsigned  n_bits=16  bin_pt=0  preci_type=Single  exp_width=8  frac_width=24  explicit_period=on  period=1  equ=P=C  opselect=C  inp2=PCIN>>17  opr=+  inp1=P  carry=CIN  dbl_ovrd=off  block_type=constant
  Delay1 : xbsIndex_r4/Delay  rst=off  infoeditControl=Selection of Reset will increase slice count due to use of real FFs and instead of SRLs  en=off  latency=1  reg_retiming=on  dbl_ovrd=off  block_type=delay
      settings: block_version=11.4
  Delay3 : xbsIndex_r4/Delay  rst=off  infoeditControl=Selection of Reset will increase slice count due to use of real FFs and instead of SRLs  en=off  latency=1  reg_retiming=on  dbl_ovrd=off  block_type=delay
      settings: block_version=11.4
  Logical1 : xbsIndex_r4/Logical  logical_function=AND  inputs=2  en=off  latency=0  precision=Full  arith_type=Unsigned  n_bits=8  bin_pt=2  align_bp=on  dbl_ovrd=off  block_type=logical
      settings: xl_area=[0, 0, 0, 0, 0, 0, 0]
  Logical2 : xbsIndex_r4/Logical  logical_function=AND  inputs=2  en=off  latency=0  precision=Full  arith_type=Unsigned  n_bits=8  bin_pt=2  align_bp=on  dbl_ovrd=off  block_type=logical
      settings: xl_area=[0, 0, 0, 0, 0, 0, 0]
  Logical3 : xbsIndex_r4/Logical  logical_function=OR  inputs=2  en=off  latency=0  precision=Full  arith_type=Unsigned  n_bits=8  bin_pt=2  align_bp=on  dbl_ovrd=off  block_type=logical
      settings: xl_area=[0, 0, 0, 0, 0, 0, 0]
  Logical4 : xbsIndex_r4/Logical  logical_function=AND  inputs=2  en=off  latency=0  precision=Full  arith_type=Unsigned  n_bits=8  bin_pt=2  align_bp=on  dbl_ovrd=off  block_type=logical
      settings: xl_area=[0, 0, 0, 0, 0, 0, 0]
  Register1 : xbsIndex_r4/Register  init=0  rst=on  en=on  dbl_ovrd=off  block_type=register
  Register3 : xbsIndex_r4/Register  init=0  rst=on  en=on  dbl_ovrd=off  block_type=register
  Relational1 : xbsIndex_r4/Relational  mode=a=b  op_type=Bool  en=off  latency=0  dbl_ovrd=off  block_type=relational
      settings: xl_area=[0, 0, 0, 0, 0, 0, 0]  block_version=10.1.3
  Relational2 : xbsIndex_r4/Relational  mode=a<b  op_type=Bool  en=off  latency=0  dbl_ovrd=off  block_type=relational
      settings: xl_area=[0, 0, 0, 0, 0, 0, 0]  block_version=10.1.3
  assert_data : xbsIndex_r4/Assert  assert_type=on  type_source=Explicitly  gui_display_data_type=Fixed-point  arith_type=Unsigned  n_bits=spead_msw  bin_pt=0  preci_type=Single  exp_width=8  frac_width=24  assert_rate=off  rate_source=Explicitly  period=1  output_port=on  block_type=assert
  data_ctr : xbsIndex_r4/Counter  cnt_type=Free Running  cnt_to=4  operation=Up  start_count=0  cnt_by_val=1  arith_type=Unsigned  n_bits=max_pkt_len_bits + 1  bin_pt=0  load_pin=off  rst=on  en=on  explicit_period=on  period=1  use_behavioral_HDL=off  implementation=Fabric  use_rpm=on  dbl_ovrd=off  block_type=counter
      settings: xl_area=[0, 0, 0, 0, 0, 0, 0]
  delay_data : xbsIndex_r4/Delay  rst=off  infoeditControl=Selection of Reset will increase slice count due to use of real FFs and instead of SRLs  en=off  latency=8  reg_retiming=on  dbl_ovrd=off  block_type=delay
      settings: block_version=11.4
  delay_data1 : xbsIndex_r4/Delay  rst=off  infoeditControl=Selection of Reset will increase slice count due to use of real FFs and instead of SRLs  en=off  latency=1  reg_retiming=on  dbl_ovrd=off  block_type=delay
      settings: block_version=11.4
  delay_data2 : xbsIndex_r4/Delay  rst=off  infoeditControl=Selection of Reset will increase slice count due to use of real FFs and instead of SRLs  en=off  latency=1  reg_retiming=on  dbl_ovrd=off  block_type=delay
      settings: block_version=11.4
  delay_valid : xbsIndex_r4/Delay  rst=off  infoeditControl=Selection of Reset will increase slice count due to use of real FFs and instead of SRLs  en=off  latency=8  reg_retiming=on  dbl_ovrd=off  block_type=delay
      settings: block_version=11.4
  edge_detect1 : casper_library_misc/edge_detect  edge=Rising  polarity=Active High  x_in=[0 0.08 0.08 0.16 0.16 0.24 0.24 0.32 0.32 0.4]  y_in="[-1 -1  1  1  1  1  1  1  1  1]"  x_out=[0.6 0.68 0.68 0.76 0.76 0.84 0.84 0.92 0.92 1]  y_out="[-1 -1  1  1 -1 -1 -1 -1 -1 -1]"
  edge_detect2 : casper_library_misc/edge_detect  edge=Rising  polarity=Active High  x_in=[0 0.08 0.08 0.16 0.16 0.24 0.24 0.32 0.32 0.4]  y_in="[-1 -1  1  1  1  1  1  1  1  1]"  x_out=[0.6 0.68 0.68 0.76 0.76 0.84 0.84 0.92 0.92 1]  y_out="[-1 -1  1  1 -1 -1 -1 -1 -1 -1]"
  hdr_ctr : xbsIndex_r4/Counter  cnt_type=Count Limited  cnt_to=8  operation=Up  start_count=0  cnt_by_val=1  arith_type=Unsigned  n_bits=4  bin_pt=0  load_pin=off  rst=on  en=on  explicit_period=on  period=1  use_behavioral_HDL=off  implementation=Fabric  use_rpm=on  dbl_ovrd=off  block_type=counter
      settings: xl_area=[0, 0, 0, 0, 0, 0, 0]
  hdra_{1..4} (4 alike) : xbsIndex_r4/Assert  assert_type=on  type_source=Explicitly  gui_display_data_type=Fixed-point  arith_type=Unsigned  n_bits=spead_lsw  bin_pt=0  preci_type=Single  exp_width=8  frac_width=24  assert_rate=off  rate_source=Explicitly  period=1  output_port=on  block_type=assert
  hdrd_1 : xbsIndex_r4/Delay  rst=off  infoeditControl=Selection of Reset will increase slice count due to use of real FFs and instead of SRLs  en=off  latency=2  reg_retiming=on  dbl_ovrd=off  block_type=delay
  hdrd_2 : xbsIndex_r4/Delay  rst=off  infoeditControl=Selection of Reset will increase slice count due to use of real FFs and instead of SRLs  en=off  latency=3  reg_retiming=on  dbl_ovrd=off  block_type=delay
  hdrd_3 : xbsIndex_r4/Delay  rst=off  infoeditControl=Selection of Reset will increase slice count due to use of real FFs and instead of SRLs  en=off  latency=4  reg_retiming=on  dbl_ovrd=off  block_type=delay
  hdrd_4 : xbsIndex_r4/Delay  rst=off  infoeditControl=Selection of Reset will increase slice count due to use of real FFs and instead of SRLs  en=off  latency=5  reg_retiming=on  dbl_ovrd=off  block_type=delay
  header_4cast4 : xbsIndex_r4/Convert  gui_display_data_type=Fixed-point  arith_type=Unsigned  n_bits=spead_lsw - 3  bin_pt=0  float_type=Single  exp_bits=8  fraction_bits=24  quantization=Truncate  overflow=Wrap  en=off  latency=1  pipeline=on  dbl_ovrd=off  block_type=convert
  header_4cat4 : xbsIndex_r4/Concat  num_inputs=2  dbl_ovrd=off  block_type=concat
  header_4const4 : xbsIndex_r4/Constant  const=0  gui_display_data_type=Fixed-point  arith_type=Unsigned  n_bits=3  bin_pt=0  preci_type=Single  exp_width=8  frac_width=24  explicit_period=off  period=1  equ=P=C  opselect=C  inp2=PCIN>>17  opr=+  inp1=P  carry=CIN  dbl_ovrd=off  block_type=constant
  header_assert{1..4} (4 alike) : xbsIndex_r4/Assert  assert_type=on  type_source=Explicitly  gui_display_data_type=Fixed-point  arith_type=Unsigned  n_bits=spead_msw  bin_pt=0  preci_type=Single  exp_width=8  frac_width=24  assert_rate=off  rate_source=Explicitly  period=1  output_port=on  block_type=assert
  header_cat{1..4} (4 alike) : xbsIndex_r4/Concat  num_inputs=2  dbl_ovrd=off  block_type=concat
  header_const{1..4} (4 alike) : xbsIndex_r4/Constant  const=65535  gui_display_data_type=Fixed-point  arith_type=Unsigned  n_bits=spead_msw - spead_lsw  bin_pt=0  preci_type=Single  exp_width=8  frac_width=24  explicit_period=off  period=1  equ=P=C  opselect=C  inp2=PCIN>>17  opr=+  inp1=P  carry=CIN  dbl_ovrd=off  block_type=constant
  heap_addr_width : xbsIndex_r4/Constant  const=spead_lsw/8  gui_display_data_type=Fixed-point  arith_type=Unsigned  n_bits=8  bin_pt=0  preci_type=Single  exp_width=8  frac_width=24  explicit_period=on  period=1  equ=P=C  opselect=C  inp2=PCIN>>17  opr=+  inp1=P  carry=CIN  dbl_ovrd=off  block_type=constant
  item_id_width : xbsIndex_r4/Constant  const=(spead_msw-spead_lsw)/8  gui_display_data_type=Fixed-point  arith_type=Unsigned  n_bits=8  bin_pt=0  preci_type=Single  exp_width=8  frac_width=24  explicit_period=on  period=1  equ=P=C  opselect=C  inp2=PCIN>>17  opr=+  inp1=P  carry=CIN  dbl_ovrd=off  block_type=constant
  mainmux : xbsIndex_r4/Mux  inputs=9  en=off  latency=1  precision=Full  arith_type="Signed  (2's comp)"  n_bits=8  bin_pt=2  quantization=Truncate  overflow=Wrap  dbl_ovrd=off  block_type=mux
      settings: xl_area=[0, 0, 0, 0, 0, 0, 0]
  num_headers : xbsIndex_r4/Constant  const=8  gui_display_data_type=Fixed-point  arith_type=Unsigned  n_bits=4  bin_pt=0  preci_type=Single  exp_width=8  frac_width=24  explicit_period=on  period=1  equ=P=C  opselect=C  inp2=PCIN>>17  opr=+  inp1=P  carry=CIN  dbl_ovrd=off  block_type=constant
  num_item_pts : xbsIndex_r4/Constant  const=7  gui_display_data_type=Fixed-point  arith_type=Unsigned  n_bits=16  bin_pt=0  preci_type=Single  exp_width=8  frac_width=24  explicit_period=on  period=1  equ=P=C  opselect=C  inp2=PCIN>>17  opr=+  inp1=P  carry=CIN  dbl_ovrd=off  block_type=constant
  only_one : xbsIndex_r4/Constant  const=1  gui_display_data_type=Fixed-point  arith_type=Unsigned  n_bits=1  bin_pt=0  preci_type=Single  exp_width=8  frac_width=24  explicit_period=on  period=1  equ=P=C  opselect=C  inp2=PCIN>>17  opr=+  inp1=P  carry=CIN  dbl_ovrd=off  block_type=constant
  data_out : Outport  VectorParamsAs1DForOutWhenUnconnected=off
  valid_out : Outport  Port=2  VectorParamsAs1DForOutWhenUnconnected=off
  eof : Outport  Port=3  VectorParamsAs1DForOutWhenUnconnected=off
  data_overflow : Outport  Port=4  VectorParamsAs1DForOutWhenUnconnected=off
  wires:
  Logical4/1 -> data_overflow/1  "overflow"
  [new_sync] -> Logical4/2
  delay_data2/1 -> delay_valid/1
  delay_data1/1 -> delay_data/1
  Logical2/1 -> [new_sync]  "new_sync"
  edge_detect2/1 -> Register1/2, Logical2/2
  Register1/1 -> Logical2/1  "armed"
  Delay3/1 -> eof/1  "eof_out"
  Relational1/1 -> Delay3/1  "eof_real"
  AddSub/1 -> Relational1/2
  data_ctr/1 -> Relational1/1  "data_ctr"
  [new_sync] -> data_ctr/1
  [writing_pld] -> data_ctr/2
  edge_detect1/1 -> Register3/2  "rst"
  num_item_pts/1 -> Concat/6
  Assert18/1 -> data_out/1
  Assert17/1 -> mainmux/2
  [pkt_data] -> assert_data/1
  Logical1/1 -> [writing_header]  "w_hdr"
  Relational2/1 -> Logical1/1  "wr_header"
  Register3/1 -> Logical1/2  "armed"
  [new_sync] -> Register3/1, Register3/3
  Delay1/1 -> valid_out/1  "valid"
  Assert7/1 -> delay_data2/1, edge_detect2/1  "data64_valid"
  data64_valid/1 -> Assert7/1
  [writing_pld] -> Logical3/2
  [writing_header] -> Logical3/1
  Logical3/1 -> Delay1/1, Logical4/1  "busy"
  [new_sync] -> hdr_ctr/1
  [writing_header] -> hdr_ctr/2
  num_headers/1 -> Relational2/2
  data64_ready/1 -> Assert5/1
  Assert5/1 -> Register1/1, Register1/3  "data64_rdy"
  Assert6/1 -> delay_data1/1  "data64"
  data64/1 -> Assert6/1
  [output_select] -> mainmux/1
  hdr_ctr/1 -> [output_select], Relational2/1  "output_sel"
  mainmux/1 -> Assert18/1  "dout"
  Constant7/1 -> Concat/5
  heap_addr_width/1 -> Concat/4
  item_id_width/1 -> Concat/3
  Constant4/1 -> Concat/2
  Constant3/1 -> Concat/1
  Concat/1 -> Assert17/1  "spd_hdr"
  delay_data/1 -> [pkt_data]  "d64"
  delay_valid/1 -> [writing_pld], edge_detect1/1  "wr_pld"
  only_one/1 -> AddSub/2
  [hdr_4] -> AddSub/1
